simulink model "heli_q8_lab2"  (R2020b)
settings: Solver=ode1  StartTime=0.0  StopTime=60  FixedStep=0.002  RelTol=1e-3  EnableMultiTasking=on
PostLoadFcn:
  | qc_set_target_type(getConfigSet(bdroot, 'QUARC Default Target Configuration'));
undefined symbols (not defined in the file or in its folder): A, B, elev_ref, F, HIL, Joystick_gain_x, Joystick_gain_y, K, qc_get_step_size, V_s0
libraries: quarc_library x4
settings Model: SimulationMode=external  ExtModeTrigDuration=5000  Creator=Rchan  LastModifiedBy=michabi
settings SolverCC: PositivePriorityOrder=on
settings DataIOCC: LimitDataPoints=on  SaveFormat=Array  SignalLoggingSaveFormat=ModelDataLogs  ReturnWorkspaceOutputs=off
settings OptimizationCC: ExpressionDepthLimit=2147483647  InitFltsAndDblsToZero=on  LifeSpan=inf
settings DebuggingCC: SaveWithParameterizedLinksMsg=none  UnderspecifiedInitializationDetection=Classic  MergeDetectMultiDrivingBlocksExec=none  SolverPrmCheckMsg=warning  MultiTaskDSMMsg=warning  MultiTaskCondExecSysMsg=none  FcnCallInpInsideContextMsg=warning  AllowSymbolicDim=off  StateNameClashWarn=warning  SFUnexpectedBacktrackingDiag=warning  SFNoUnconditionalDefaultTransitionDiag=warning  SFExecutionAtInitializationDiag=none  ArithmeticOperatorsInVariantConditions=warning
settings HardwareCC: ProdBitPerPointer=32  ProdBitPerSizeT=32  ProdBitPerPtrDiffT=32  ProdLargestAtomicFloat=None  ProdIntDivRoundTo=Undefined  ProdEndianess=Unspecified  ProdWordSize=32  ProdHWDeviceType=32-bit Generic
settings ModelReferenceCC: PropagateSignalLabelsOutOfModel=off
settings SFSimCC: SimUseLocalCustomCode=off  CustomCodeUndefinedFunction=UseInterfaceOnly
settings RTWCC: Description=QUARC Win64 Target  SystemTargetFile=quarc_win64.tlc  TemplateMakefile=quarc_default_tmf  RTWUseLocalCustomCode=off
settings CodeAppCC: StateflowObjectComments=on
settings GRTTargetCC: TargetLangStandard=C89/C90 (ANSI)  ParMdlRefBuildCompliant=off  CompOptLevelCompliant=off  CombineOutputUpdateFcns=off  MatFileLogging=off  GRTInterface=on  UseToolchainInfoCompliant=off  ExtMode=on  ExtModeMexFile=quarc_comm
settings ConfigComp: CovMetricSettings=dw  CovSaveCumulativeToWorkspaceVar=on  CovSaveSingleToWorkspaceVar=on  CovExternalEMLEnable=off  CovSFcnEnable=off

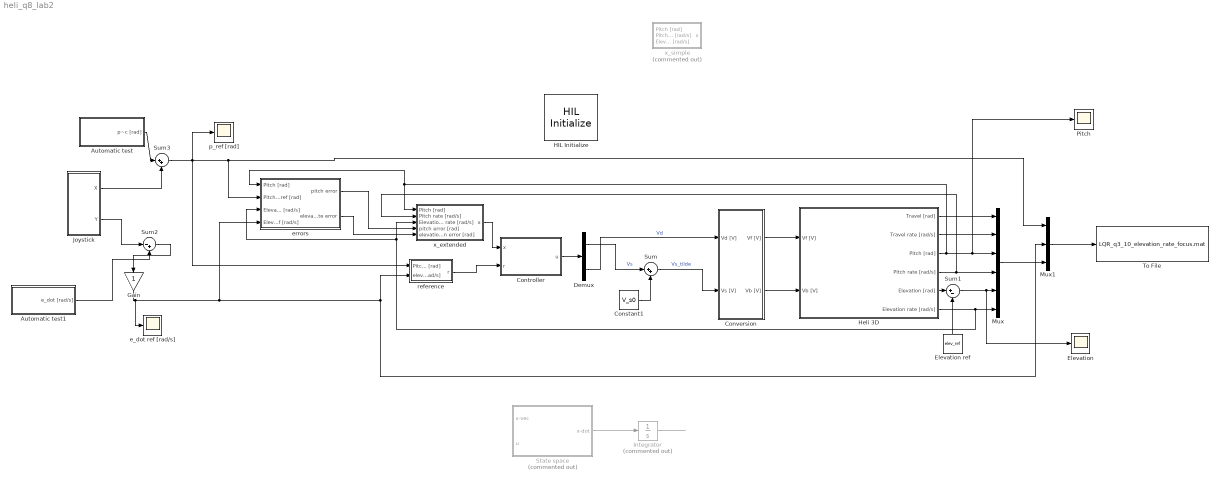
== system heli_q8_lab2 ==
  Automatic test : Subsystem
  Automatic test1 : Subsystem
  Constant1 : Constant  Value=V_s0
  Controller : Subsystem
  Conversion : Subsystem
  Demux : Demux  Outputs=2
  Elevation : Scope
  Elevation ref : Constant  Value=elev_ref
  Gain : Gain
  HIL Initialize : quarc_library/Data Acquisition/Generic/Configuration/HIL Initialize  Priority=-99  object_name=HIL-1  board_type=q8_usb  board_number=0  board_options=update_rate=normal;decimation=1  exclusive=off  active=off  hardware_clocks=[0:2]  clock_modes=[]  initial_clock_frequencies=[]  set_clock_params_at_start=off  set_clock_params_at_switch_in=off  set_clock_frequencies_at_start=off  set_clock_frequencies_at_switch_in=off  analog_input_channels=[0:7]  analog_input_configurations=[]  analog_input_maximums=10  analog_input_minimums=-10  set_analog_input_params_at_start=on  set_analog_input_params_at_switch_in=off  analog_output_channels=[0:7]  analog_output_maximums=10  analog_output_minimums=-10  initial_analog_outputs=[0]  final_analog_outputs=[0]  watchdog_analog_outputs=0  set_analog_output_params_at_start=on  set_analog_output_params_at_switch_in=off  set_analog_outputs_at_start=on  set_analog_outputs_at_switch_in=off  set_analog_outputs_at_terminate=on  set_analog_outputs_at_switch_out=off  set_analog_outputs_on_watchdog=off  digital_input_channels=[]  digital_output_channels=[]  digital_output_configuration=[]  initial_digital_outputs=[1]  final_digital_outputs=[1]  watchdog_digital_outputs=[1]  set_digital_output_params_at_start=off  set_digital_output_params_at_switch_in=off  set_digital_outputs_at_start=on  set_digital_outputs_at_switch_in=off  set_digital_outputs_at_terminate=on  set_digital_outputs_at_switch_out=off  set_digital_outputs_on_watchdog=off  encoder_channels=[0:7]  quadrature=[4]  encoder_filter_frequency=[]  initial_encoder_counts=[0]  set_encoder_params_at_start=on  set_encoder_params_at_switch_in=off  set_encoder_counts_at_start=on  set_encoder_counts_at_switch_in=off  pwm_channels=[0:7]  pwm_modes=0  pwm_frequency=99.532799999999995e6/4095  pwm_configuration=[0]  pwm_alignment=[0]  pwm_polarity=[1]  pwm_leading_deadband=[0]  pwm_trailing_deadband=[0]  initial_pwm_outputs=[0]  final_pwm_outputs=[0]  watchdog_pwm_outputs=[0]  set_pwm_params_at_start=on  set_pwm_params_at_switch_in=off  set_pwm_outputs_at_start=on  set_pwm_outputs_at_switch_in=off  set_pwm_outputs_at_terminate=on  set_pwm_outputs_at_switch_out=off  set_pwm_outputs_on_watchdog=off  other_output_channels=[]  initial_other_outputs=[]  final_other_outputs=[]  watchdog_other_outputs=[]  set_other_outputs_at_start=off  set_other_outputs_at_switch_in=off  set_other_outputs_at_terminate=off  set_other_outputs_at_switch_out=off  set_other_outputs_on_watchdog=off
  Heli 3D : Subsystem
  Integrator : Integrator  Commented=on
  Joystick : Subsystem
  Mux : Mux  Inputs=6
  Mux1 : Mux  Inputs=3
  Pitch : Scope
  State space : Subsystem  Commented=on
  Sum : Sum  Inputs=|++
  Sum1 : Sum  Inputs=|+-
  Sum2 : Sum  Inputs=|-+
  Sum3 : Sum  Inputs=|++
  To File : ToFile  Filename=LQR_q3_10_elevation_rate_focus.mat
  e_dot ref [rad/s] : Scope
  errors : Subsystem
  p_ref [rad] : Scope
  reference : Subsystem
  x_extended : Subsystem
  x_simple : Subsystem  Commented=on
  wires:
  Conversion/2(Vb [V]) -> Heli 3D/2(Vb [V])
  Conversion/1(Vf [V]) -> Heli 3D/1(Vf [V])
  Heli 3D/1(Travel [rad]) -> Mux/1
  Heli 3D/2(Travel rate [rad/s]) -> Mux/2
  Heli 3D/3(Pitch [rad]) -> errors/1(Pitch [rad]), x_extended/1(Pitch [rad]), Pitch/1, Mux/3
  Heli 3D/4(Pitch rate [rad/s]) -> x_extended/2(Pitch rate [rad/s]), Mux/4
  Heli 3D/6(Elevation rate [rad/s]) -> errors/3(Elevation rate [rad/s]), x_extended/3(Elevation rate [rad/s]), Mux/6
  Heli 3D/5(Elevation [rad]) -> Sum1/1
  Constant1/1 -> Sum/2
  Sum/1 -> Conversion/2(Vs [V])  "Vs_tilde"
  Gain/1 -> e_dot ref [rad/s]/1, errors/4(Elevation rate ref [rad/s]), reference/2(elevation rate [rad/s]), Mux1/2
  Joystick/1(X) -> Sum3/2
  Sum1/1 -> Elevation/1, Mux/5
  Elevation ref/1 -> Sum1/2
  Mux/1 -> Mux1/3
  Integrator/1 -> ?
  State space/1(x-dot) -> Integrator/1
  Demux/1 -> Sum/1  "Vs"
  Demux/2 -> Conversion/1(Vd [V])  "Vd"
  Mux1/1 -> To File/1
  Automatic test1/1(e_dot [rad/s]) -> Sum2/2
  Joystick/2(Y) -> Sum2/1
  Sum2/1 -> Gain/1
  Controller/1(u) -> Demux/1
  x_extended/1(x) -> Controller/1(x)
  reference/1(r) -> Controller/2(r)
  Automatic test/1(p~c [rad]) -> Sum3/1
  Sum3/1 -> Mux1/1, errors/2(Pitch ref [rad]), reference/1(Pitch [rad]), p_ref [rad]/1
  errors/1(pitch error) -> x_extended/4(pitch error [rad])
  errors/2(elevation rate error) -> x_extended/5(elevation error [rad])

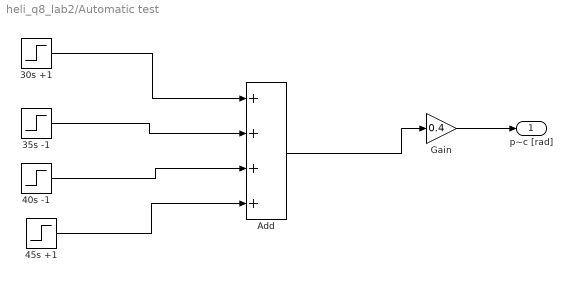
== system heli_q8_lab2/Automatic test ==
  30s +1 : Step  Time=30  SampleTime=0
  35s -1 : Step  Time=35  After=-1  SampleTime=0
  40s -1 : Step  Time=40  After=-1  SampleTime=0
  45s +1 : Step  Time=45  SampleTime=0
  Add : Sum  Inputs=++++
  Gain : Gain  Gain=0.4
  p~c [rad] : Outport
  wires:
  30s +1/1 -> Add/1
  Add/1 -> Gain/1
  35s -1/1 -> Add/2
  40s -1/1 -> Add/3
  45s +1/1 -> Add/4
  Gain/1 -> p~c [rad]/1

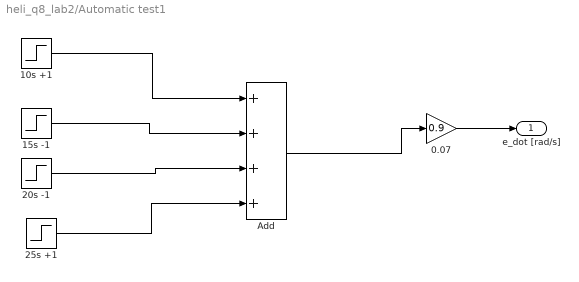
== system heli_q8_lab2/Automatic test1 ==
  0.07 : Gain  Gain=0.9
  10s +1 : Step  Time=10  SampleTime=0
  15s -1 : Step  Time=15  After=-1  SampleTime=0
  20s -1 : Step  Time=20  After=-1  SampleTime=0
  25s +1 : Step  Time=25  SampleTime=0
  Add : Sum  Inputs=++++
  e_dot [rad/s] : Outport
  wires:
  10s +1/1 -> Add/1
  Add/1 -> 0.07/1
  15s -1/1 -> Add/2
  20s -1/1 -> Add/3
  25s +1/1 -> Add/4
  0.07/1 -> e_dot [rad/s]/1

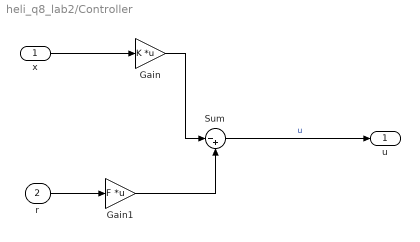
== system heli_q8_lab2/Controller ==
  x : Inport
  r : Inport  Port=2
  Gain : Gain  Gain=K  Multiplication=Matrix(K*u)
  Gain1 : Gain  Gain=F  Multiplication=Matrix(K*u)
  Sum : Sum  Inputs=|-+
  u : Outport
  wires:
  x/1 -> Gain/1
  Gain/1 -> Sum/1
  Gain1/1 -> Sum/2
  Sum/1 -> u/1  "u"
  r/1 -> Gain1/1

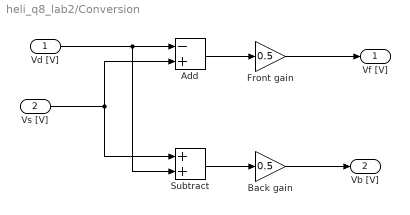
== system heli_q8_lab2/Conversion ==
  Vd [V] : Inport
  Vs [V] : Inport  Port=2
  Add : Sum  Inputs=-+
  Back gain : Gain  Gain=0.5
  Front gain : Gain  Gain=0.5
  Subtract : Sum
  Vf [V] : Outport
  Vb [V] : Outport  Port=2
  wires:
  Vd [V]/1 -> Subtract/2, Add/1
  Vs [V]/1 -> Subtract/1, Add/2
  Subtract/1 -> Back gain/1
  Back gain/1 -> Vb [V]/1
  Add/1 -> Front gain/1
  Front gain/1 -> Vf [V]/1

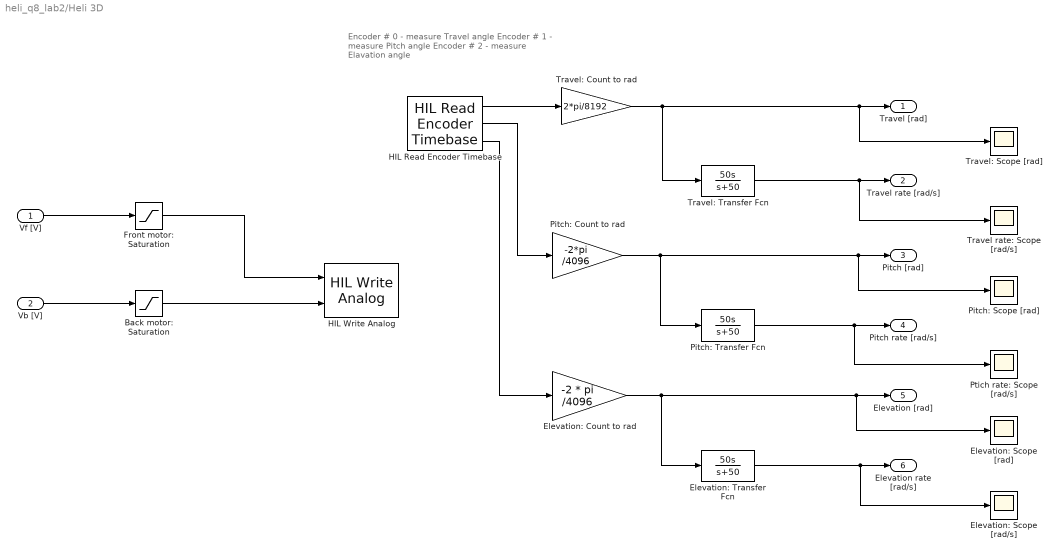
== system heli_q8_lab2/Heli 3D ==
  note: Encoder # 0 - measure Travel angle
      | Encoder # 1 - measure Pitch angle
      | Encoder # 2 - measure Elavation angle
  Vf [V] : Inport
  Vb [V] : Inport  Port=2
  Back motor: Saturation : Saturate  UpperLimit=5  LowerLimit=-5
  Elevation: Count to rad : Gain  Gain=-2 * pi /4096
  Elevation: Scope [rad/s] : Scope
  Elevation: Scope [rad] : Scope
  Elevation: Transfer Fcn : TransferFcn  Numerator=[50 0]  Denominator=[1 50]
  Front motor: Saturation : Saturate  UpperLimit=5  LowerLimit=-5
  HIL Read Encoder Timebase : quarc_library/Data Acquisition/Generic/Timebases/HIL Read Encoder Timebase  object_name=HIL-1  clock=0  channels=[0:2]  active=on  vector_output=off  data_type_mode=Inherit via back propagation  data_type=double  overflow_mode=Error on overflow  samples_in_buffer=max(ceil(1/qc_get_step_size), 1)
  HIL Write Analog : quarc_library/Data Acquisition/Generic/Immediate I//O/HIL Write Analog  object_name=HIL-1  channels=[0:1]  sample_time=-1  active=off  vector_input=off
  Pitch: Count to rad : Gain  Gain=-2*pi /4096
  Pitch: Scope [rad] : Scope
  Pitch: Transfer Fcn : TransferFcn  Numerator=[50 0]  Denominator=[1 50]
  Ptich rate: Scope [rad/s] : Scope
  Travel rate: Scope [rad/s] : Scope
  Travel: Count to rad : Gain  Gain=2*pi/8192
  Travel: Scope [rad] : Scope
  Travel: Transfer Fcn : TransferFcn  Numerator=[50 0]  Denominator=[1 50]
  Travel [rad] : Outport
  Travel rate [rad/s] : Outport  Port=2
  Pitch [rad] : Outport  Port=3
  Pitch rate [rad/s] : Outport  Port=4
  Elevation [rad] : Outport  Port=5
  Elevation rate [rad/s] : Outport  Port=6
  wires:
  HIL Read Encoder Timebase/1 -> Travel: Count to rad/1
  HIL Read Encoder Timebase/2 -> Pitch: Count to rad/1
  HIL Read Encoder Timebase/3 -> Elevation: Count to rad/1
  Travel: Count to rad/1 -> Travel: Scope [rad]/1, Travel [rad]/1, Travel: Transfer Fcn/1
  Travel: Transfer Fcn/1 -> Travel rate: Scope [rad/s]/1, Travel rate [rad/s]/1
  Pitch: Count to rad/1 -> Pitch: Transfer Fcn/1, Pitch: Scope [rad]/1, Pitch [rad]/1
  Pitch: Transfer Fcn/1 -> Ptich rate: Scope [rad/s]/1, Pitch rate [rad/s]/1
  Elevation: Count to rad/1 -> Elevation: Transfer Fcn/1, Elevation: Scope [rad]/1, Elevation [rad]/1
  Elevation: Transfer Fcn/1 -> Elevation: Scope [rad/s]/1, Elevation rate [rad/s]/1
  Vf [V]/1 -> Front motor: Saturation/1
  Vb [V]/1 -> Back motor: Saturation/1
  Front motor: Saturation/1 -> HIL Write Analog/1
  Back motor: Saturation/1 -> HIL Write Analog/2

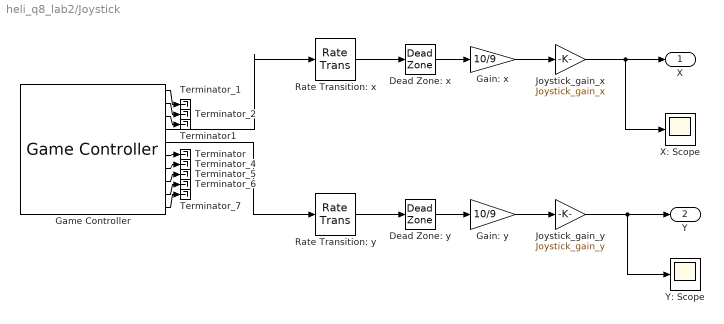
== system heli_q8_lab2/Joystick ==
  Dead Zone: x : DeadZone  LowerValue=-0.1  UpperValue=0.1  SaturateOnIntegerOverflow=on
  Dead Zone: y : DeadZone  LowerValue=-0.1  UpperValue=0.1  SaturateOnIntegerOverflow=on
  Gain: x : Gain  Gain=10/9
  Gain: y : Gain  Gain=10/9
  Game Controller : quarc_library/Devices/Peripherals/Target/Game Controller  controller=1  buffer_size=12  deadzone=[]  saturation=[]  sample_time=max(qc_get_step_size, 0.01)  auto_center=off  enabled=on
      settings: SourceProductName=QUARC Targets
  Joystick_gain_x : Gain  Gain=Joystick_gain_x
  Joystick_gain_y : Gain  Gain=Joystick_gain_y
  Rate Transition: x : RateTransition
  Rate Transition: y : RateTransition
  Terminator : Terminator
  Terminator1 : Terminator
  Terminator_{1..2,4..7} (6 alike) : Terminator
  X: Scope : Scope
  Y: Scope : Scope
  X : Outport
  Y : Outport  Port=2
  wires:
  Rate Transition: y/1 -> Dead Zone: y/1
  Rate Transition: x/1 -> Dead Zone: x/1
  Game Controller/5 -> Rate Transition: y/1
  Game Controller/4 -> Rate Transition: x/1
  Game Controller/1 -> Terminator_1/1
  Game Controller/2 -> Terminator_2/1
  Game Controller/7 -> Terminator_4/1
  Game Controller/8 -> Terminator_5/1
  Game Controller/9 -> Terminator_6/1
  Game Controller/10 -> Terminator_7/1
  Game Controller/3 -> Terminator1/1
  Game Controller/6 -> Terminator/1
  Dead Zone: x/1 -> Gain: x/1
  Dead Zone: y/1 -> Gain: y/1
  Gain: x/1 -> Joystick_gain_x/1
  Gain: y/1 -> Joystick_gain_y/1
  Joystick_gain_x/1 -> X/1, X: Scope/1
  Joystick_gain_y/1 -> Y: Scope/1, Y/1

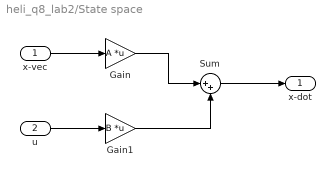
== system heli_q8_lab2/State space ==
  x-vec : Inport
  u : Inport  Port=2
  Gain : Gain  Gain=A  Multiplication=Matrix(K*u)
  Gain1 : Gain  Gain=B  Multiplication=Matrix(K*u)
  Sum : Sum  Inputs=|++
  x-dot : Outport
  wires:
  x-vec/1 -> Gain/1
  u/1 -> Gain1/1
  Gain/1 -> Sum/1
  Gain1/1 -> Sum/2
  Sum/1 -> x-dot/1

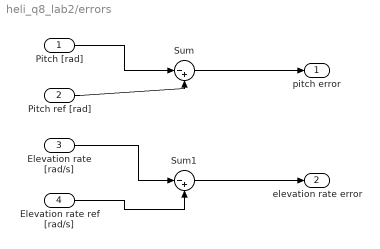
== system heli_q8_lab2/errors ==
  Pitch [rad] : Inport
  Pitch ref [rad] : Inport  Port=2
  Elevation rate [rad/s] : Inport  Port=3
  Elevation rate ref [rad/s] : Inport  Port=4
  Sum : Sum  Inputs=|-+
  Sum1 : Sum  Inputs=|-+
  pitch error : Outport
  elevation rate error : Outport  Port=2
  wires:
  Pitch [rad]/1 -> Sum/1
  Elevation rate ref [rad/s]/1 -> Sum1/2
  Sum/1 -> pitch error/1
  Sum1/1 -> elevation rate error/1
  Pitch ref [rad]/1 -> Sum/2
  Elevation rate [rad/s]/1 -> Sum1/1

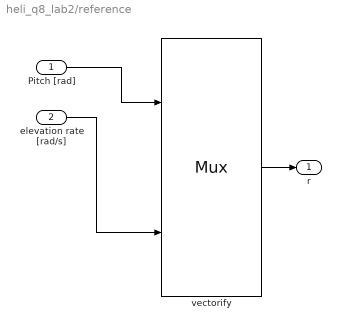
== system heli_q8_lab2/reference ==
  Pitch [rad] : Inport
  elevation rate [rad/s] : Inport  Port=2
  vectorify : Mux  Inputs=2
  r : Outport
  wires:
  Pitch [rad]/1 -> vectorify/1
  elevation rate [rad/s]/1 -> vectorify/2
  vectorify/1 -> r/1

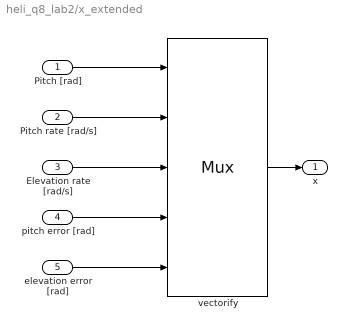
== system heli_q8_lab2/x_extended ==
  Pitch [rad] : Inport
  Pitch rate [rad/s] : Inport  Port=2
  Elevation rate [rad/s] : Inport  Port=3
  pitch error [rad] : Inport  Port=4
  elevation error [rad] : Inport  Port=5
  vectorify : Mux  Inputs=5
  x : Outport
  wires:
  Pitch [rad]/1 -> vectorify/1
  Pitch rate [rad/s]/1 -> vectorify/2
  Elevation rate [rad/s]/1 -> vectorify/3
  vectorify/1 -> x/1
  pitch error [rad]/1 -> vectorify/4
  elevation error [rad]/1 -> vectorify/5

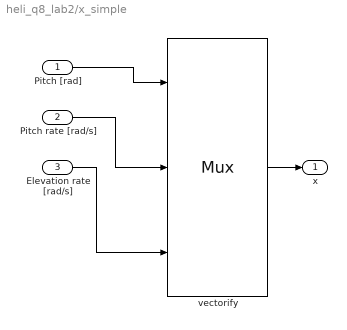
== system heli_q8_lab2/x_simple ==
  Pitch [rad] : Inport
  Pitch rate [rad/s] : Inport  Port=2
  Elevation rate [rad/s] : Inport  Port=3
  vectorify : Mux  Inputs=3
  x : Outport
  wires:
  Pitch [rad]/1 -> vectorify/1
  Pitch rate [rad/s]/1 -> vectorify/2
  Elevation rate [rad/s]/1 -> vectorify/3
  vectorify/1 -> x/1
